simulink model "MotorControl_test"  (R2013b)
settings: Solver=FixedStepDiscrete  StartTime=0.0  StopTime=10.0  FixedStep=0.05  RelTol=1e-3
InitFcn:
  | Vs = 4.5; % The supply voltage
settings Model: Creator=nding  LastModifiedBy=nding

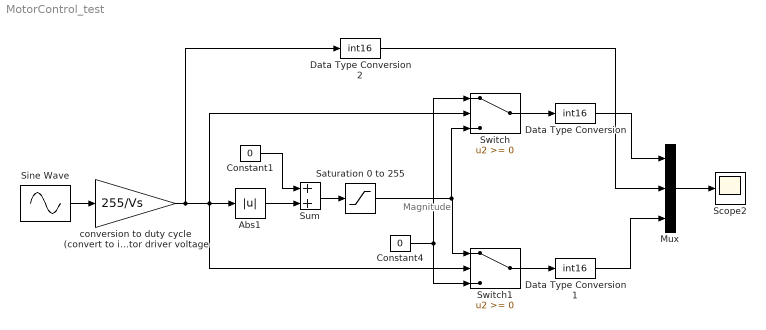
== system MotorControl_test ==
  note: Magnitude
  Abs1 : Abs
  Constant1 : Constant  Value=0
  Constant4 : Constant  Value=0
  Data Type Conversion : DataTypeConversion  OutDataTypeStr=int16
  Data Type Conversion1 : DataTypeConversion  OutDataTypeStr=int16
  Data Type Conversion2 : DataTypeConversion  OutDataTypeStr=int16
  Mux : Mux  Inputs=3
  Saturation 0 to 255 : Saturate  UpperLimit=255  LowerLimit=0
  Scope2 : Scope
      settings: SaveName=ScopeData2
  Sine Wave : Sin  Amplitude=Vs  Frequency=2*pi*0.1  SampleTime=0.05
  Sum : Sum
  Switch : Switch
  Switch1 : Switch
  conversion to duty cycle (convert to int) denominator is motor driver voltage : Gain  Gain=255/Vs  OutDataTypeStr=int16
  wires:
  Constant1/1 -> Sum/1
  Sum/1 -> Saturation 0 to 255/1
  Abs1/1 -> Sum/2
  Data Type Conversion1/1 -> Mux/3
  Switch1/1 -> Data Type Conversion1/1
  Switch/1 -> Data Type Conversion/1
  Saturation 0 to 255/1 -> Switch1/1, Switch/3
  Constant4/1 -> Switch1/3, Switch/1
  conversion to duty cycle (convert to int) denominator is motor driver voltage/1 -> Data Type Conversion2/1, Switch/2, Abs1/1, Switch1/2
  Sine Wave/1 -> conversion to duty cycle (convert to int) denominator is motor driver voltage/1
  Data Type Conversion/1 -> Mux/1
  Mux/1 -> Scope2/1
  Data Type Conversion2/1 -> Mux/2
